simulink library "mssSimulink"  (R2024a)
settings: Solver=ode45  StartTime=0.0  StopTime=10.0  RelTol=1e-3
undefined symbols (not defined in the file): ABC, CN_data, CX_data, CY_data, D, G, Hoerner, K_supply, kt2ms, MA, magnitude, MRB, pathlength, RAO_Amp, RAO_Dir, RAO_Freq, RAO_Phase, RAO_Vel, RAO_yaw_back, RAO_yaw_quant, RAO_yaw_quantization_flag, rho_a, slcm, T_supply, table, vessel, vesselABC
libraries: $bdroot x99, simulink x13
(part 5 of 9)

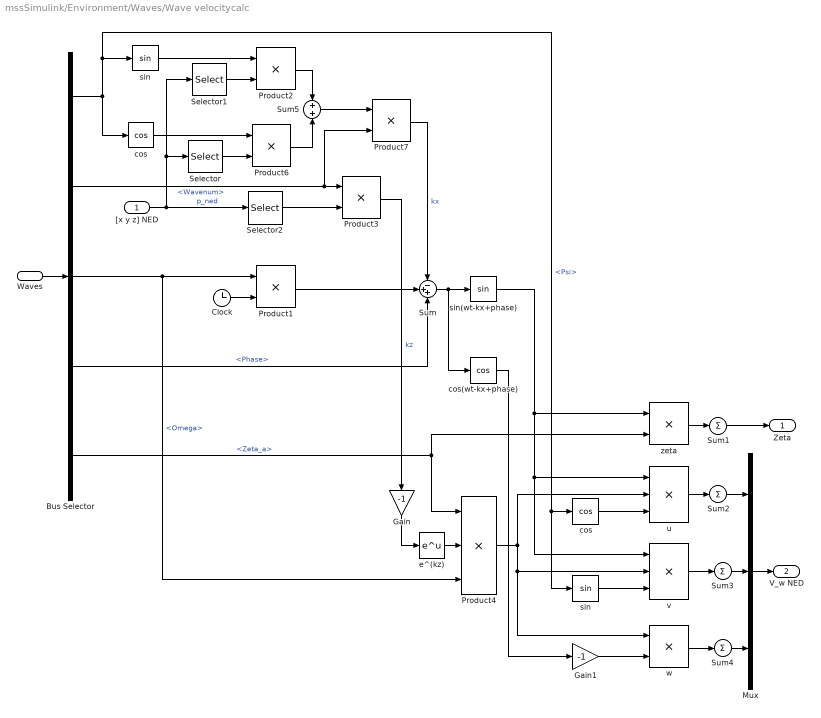
== system mssSimulink/Environment/Waves/Wave velocitycalc ==
  "[x y z] NED" : Inport
  Waves : Inport  Port=2
  Bus Selector : BusSelector  OutputSignals=Psi,Wavenum,Omega,Phase,Zeta_a
  Clock : Clock
  Gain : Gain  Gain=-1  SaturateOnIntegerOverflow=on  OutDataTypeStr=Inherit: Same as input  ParamDataTypeStr=Inherit: Same as input
  Gain1 : Gain  Gain=-1  SaturateOnIntegerOverflow=on  OutDataTypeStr=Inherit: Same as input  ParamDataTypeStr=Inherit: Same as input
  Mux : Mux  Inputs=3
  Product{1..3,6..7} (5 alike) : Product  Inputs=**  SaturateOnIntegerOverflow=on  OutDataTypeStr=Inherit: Same as first input
  Product4 : Product  Inputs=3  SaturateOnIntegerOverflow=on  OutDataTypeStr=Inherit: Same as first input
  Selector : Selector  InputPortWidth=3  IndexOptions=Index vector (dialog)  Indices=1  OutputSizes=1
  Selector1 : Selector  InputPortWidth=3  IndexOptions=Index vector (dialog)  Indices=2  OutputSizes=1
  Selector2 : Selector  InputPortWidth=3  IndexOptions=Index vector (dialog)  Indices=3  OutputSizes=1
  Sum : Sum  Inputs=-++  SaturateOnIntegerOverflow=on
  Sum{1..4} (4 alike) : Sum  Inputs=1  SaturateOnIntegerOverflow=on
  Sum5 : Sum  SaturateOnIntegerOverflow=on
  cos : Trigonometry  Operator=cos
  "cos " : Trigonometry  Operator=cos
  cos(wt-kx+phase) : Trigonometry  Operator=cos
  e^(kz) : Math  SignedPower=on
  sin : Trigonometry
  "sin " : Trigonometry
  sin(wt-kx+phase) : Trigonometry
  u : Product  Inputs=***  SaturateOnIntegerOverflow=on  OutDataTypeStr=Inherit: Same as first input
  v : Product  Inputs=***  SaturateOnIntegerOverflow=on  OutDataTypeStr=Inherit: Same as first input
  w : Product  Inputs=**  SaturateOnIntegerOverflow=on  OutDataTypeStr=Inherit: Same as first input
  zeta : Product  Inputs=**  SaturateOnIntegerOverflow=on  OutDataTypeStr=Inherit: Same as first input
  Zeta : Outport  VectorParamsAs1DForOutWhenUnconnected=off
  V_w NED : Outport  Port=2  VectorParamsAs1DForOutWhenUnconnected=off
  wires:
  Gain1/1 -> w/2
  "cos "/1 -> u/3
  "sin "/1 -> v/3
  Selector2/1 -> Product3/2
  "[x y z] NED"/1 -> Selector/1, Selector1/1, Selector2/1  "p_ned"
  Sum5/1 -> Product7/1
  Product6/1 -> Sum5/2
  Product2/1 -> Sum5/1
  sin/1 -> Product2/1
  Selector1/1 -> Product2/2
  cos/1 -> Product6/1
  Selector/1 -> Product6/2
  Bus Selector/2 -> Product3/1, Product7/2  "<Wavenum>"
  Gain/1 -> e^(kz)/1
  Bus Selector/5 -> Product4/1, zeta/2  "<Zeta_a>"
  Bus Selector/4 -> Sum/3  "<Phase>"
  Bus Selector/3 -> Product4/3, Product1/1  "<Omega>"
  Waves/1 -> Bus Selector/1
  cos(wt-kx+phase)/1 -> Gain1/1
  Product4/1 -> w/1, v/2, u/2
  e^(kz)/1 -> Product4/2
  Product7/1 -> Sum/1  "kx"
  zeta/1 -> Sum1/1
  sin(wt-kx+phase)/1 -> v/1, u/1, zeta/1
  Sum/1 -> cos(wt-kx+phase)/1, sin(wt-kx+phase)/1
  Product1/1 -> Sum/2
  Bus Selector/1 -> sin/1, "cos "/1, "sin "/1, cos/1  "<Psi>"
  Product3/1 -> Gain/1  "kz"
  Sum1/1 -> Zeta/1
  w/1 -> Sum4/1
  u/1 -> Sum2/1
  v/1 -> Sum3/1
  Sum2/1 -> Mux/1
  Sum3/1 -> Mux/2
  Sum4/1 -> Mux/3
  Mux/1 -> V_w NED/1
  Clock/1 -> Product1/2

== system mssSimulink/Environment/Waves/Waves ==
  Bus Creator : BusCreator  Inputs=5
  Omega : Constant  Value=Omega
  Phase : Constant  Value=Phase
  Psi : Constant  Value=Psi
  Wavenum : Constant  Value=Wavenum
  Zeta_a : Constant  Value=Zeta_a
  "wave direction " : Constant  Value=psi_mean
  Waves : Outport  VectorParamsAs1DForOutWhenUnconnected=off
  wave direction : Outport  Port=2  VectorParamsAs1DForOutWhenUnconnected=off
  wires:
  Phase/1 -> Bus Creator/5  "Phase"
  Psi/1 -> Bus Creator/2  "Psi"
  Omega/1 -> Bus Creator/1  "Omega"
  Bus Creator/1 -> Waves/1
  Zeta_a/1 -> Bus Creator/3  "Zeta_a"
  Wavenum/1 -> Bus Creator/4  "Wavenum"
  "wave direction "/1 -> wave direction/1

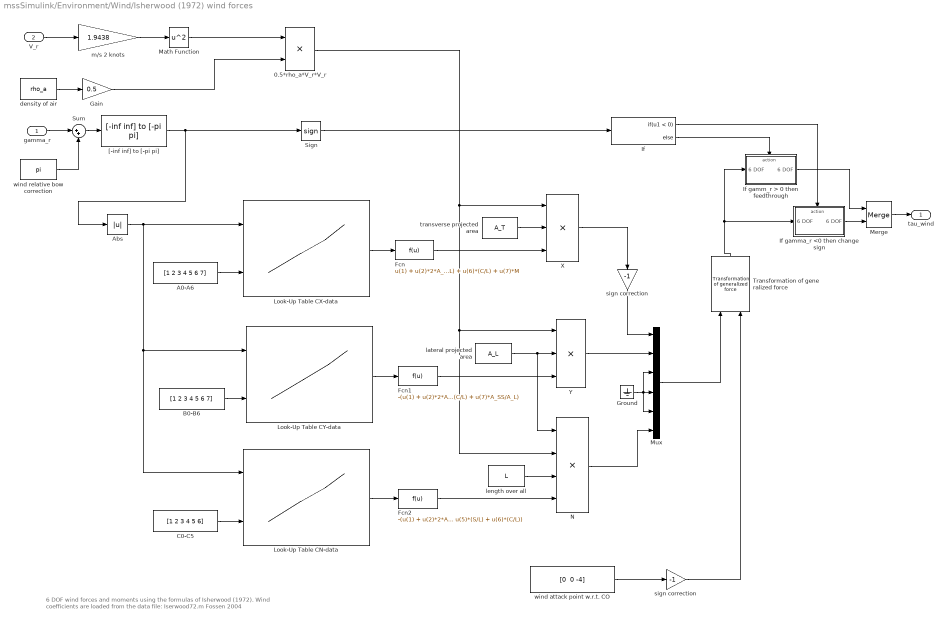
== system mssSimulink/Environment/Wind/Isherwood (1972) wind forces ==
  note: 6 DOF wind forces and moments using the formulas of Isherwood (1972).
      | Wind coefficients are loaded from the data file: Iserwood72.m
      |
      | Fossen 2004
  gamma_r : Inport
  V_r : Inport  Port=2
  0.5*rho_a*V_r*V_r : Product  SaturateOnIntegerOverflow=on  OutDataTypeStr=Inherit: Same as first input
  A0-A6 : Constant  Value=[1 2 3 4 5 6 7]
  Abs : Abs
  B0-B6 : Constant  Value=[1 2 3 4 5 6 7]
  C0-C5 : Constant  Value=[1 2 3 4 5 6]
  Fcn : Fcn  Expr=u(1) + u(2)*2*A_L/L^2 + u(3)*2*A_T/B^2 + u(4)*(L/B) + u(5)*(S/L) + u(6)*(C/L) + u(7)*M
  Fcn1 : Fcn  Expr=-(u(1) + u(2)*2*A_L/L^2 + u(3)*2*A_T/B^2 + u(4)*(L/B) + u(5)*(S/L) + u(6)*(C/L) + u(7)*A_SS/A_L)
  Fcn2 : Fcn  Expr=-(u(1) + u(2)*2*A_L/L^2 + u(3)*2*A_T/B^2 + u(4)*(L/B) + u(5)*(S/L) + u(6)*(C/L))
  Gain : Gain  Gain=0.5  SaturateOnIntegerOverflow=on  OutDataTypeStr=Inherit: Same as input  ParamDataTypeStr=Inherit: Same as input
  Ground : Ground
  If : If  IfExpression=u1 < 0
  If gamm_r > 0 then feedthrough : Subsystem  TreatAsAtomicUnit=on
  If gamma_r <0 then change sign : Subsystem  TreatAsAtomicUnit=on
  Look-Up Table CN-data : Lookup2D  RowIndex=gamma_r_iserwood  ColumnIndex=[1:6]  Table=CN_data  OutDataTypeStr=double  InputSameDT=off
  Look-Up Table CX-data : Lookup2D  RowIndex=gamma_r_iserwood  ColumnIndex=[1:7]  Table=CX_data  OutDataTypeStr=double  InputSameDT=off
  Look-Up Table CY-data : Lookup2D  RowIndex=gamma_r_iserwood  ColumnIndex=[1:7]  Table=CY_data  OutDataTypeStr=double  InputSameDT=off
  Math Function : Math  Operator=square  SignedPower=on
  Merge : Merge
  Mux : Mux  Inputs=6
  N : Product  Inputs=4  SaturateOnIntegerOverflow=on  OutDataTypeStr=Inherit: Same as first input
  Sign : Signum
  Sum : Sum  Inputs=|++  SaturateOnIntegerOverflow=on
  Transformation of gene ralized force : $bdroot/Modelling/Kinematics/Transformation of generalized force
  X : Product  Inputs=3  SaturateOnIntegerOverflow=on  OutDataTypeStr=Inherit: Same as first input
  Y : Product  Inputs=3  SaturateOnIntegerOverflow=on  OutDataTypeStr=Inherit: Same as first input
  "[-inf inf] to [-pi pi]" : $bdroot/Utilities/Math Operations/[-inf inf] to [-pi pi]
  density of air : Constant  Value=rho_a
  lateral projected area : Constant  Value=A_L
  length over all : Constant  Value=L
  m/s 2 knots : Gain  Gain=1.9438  SaturateOnIntegerOverflow=on  OutDataTypeStr=Inherit: Same as input  ParamDataTypeStr=Inherit: Same as input
  sign correction : Gain  Gain=-1  SaturateOnIntegerOverflow=on  OutDataTypeStr=Inherit: Same as input  ParamDataTypeStr=Inherit: Same as input
  "sign correction " : Gain  Gain=-1  SaturateOnIntegerOverflow=on  OutDataTypeStr=Inherit: Same as input  ParamDataTypeStr=Inherit: Same as input
  transverse projected area : Constant  Value=A_T
  wind attack point w.r.t. CO : Constant  Value="[0  0 -4]"
  wind relative bow correction : Constant  Value=pi
  tau_wind : Outport  VectorParamsAs1DForOutWhenUnconnected=off
  wires:
  A0-A6/1 -> Look-Up Table CX-data/2
  Look-Up Table CX-data/1 -> Fcn/1
  B0-B6/1 -> Look-Up Table CY-data/2
  C0-C5/1 -> Look-Up Table CN-data/2
  Look-Up Table CY-data/1 -> Fcn1/1
  Look-Up Table CN-data/1 -> Fcn2/1
  gamma_r/1 -> Sum/1
  Fcn/1 -> X/3
  Fcn1/1 -> Y/3
  Fcn2/1 -> N/4
  density of air/1 -> Gain/1
  V_r/1 -> m/s 2 knots/1
  Math Function/1 -> 0.5*rho_a*V_r*V_r/1
  Gain/1 -> 0.5*rho_a*V_r*V_r/2
  0.5*rho_a*V_r*V_r/1 -> X/1, Y/1, N/2
  transverse projected area/1 -> X/2
  X/1 -> sign correction/1
  lateral projected area/1 -> Y/2, N/1
  Y/1 -> Mux/2
  N/1 -> Mux/6
  length over all/1 -> N/3
  m/s 2 knots/1 -> Math Function/1
  Abs/1 -> Look-Up Table CX-data/1, Look-Up Table CY-data/1, Look-Up Table CN-data/1
  Transformation of gene ralized force/1 -> If gamma_r <0 then change sign/1(6 DOF), If gamm_r > 0 then feedthrough/1(6 DOF)
  If/2 -> If gamm_r > 0 then feedthrough/Action
  If/1 -> If gamma_r <0 then change sign/Action
  If gamma_r <0 then change sign/1("6 DOF  ") -> Merge/2
  If gamm_r > 0 then feedthrough/1("6 DOF  ") -> Merge/1
  Sign/1 -> If/1
  wind attack point w.r.t. CO/1 -> "sign correction "/1
  "sign correction "/1 -> Transformation of gene ralized force/2
  Merge/1 -> tau_wind/1
  Mux/1 -> Transformation of gene ralized force/1
  Ground/1 -> Mux/3, Mux/4, Mux/5
  wind relative bow correction/1 -> Sum/2
  Sum/1 -> "[-inf inf] to [-pi pi]"/1
  "[-inf inf] to [-pi pi]"/1 -> Abs/1, Sign/1
  sign correction/1 -> Mux/1

== system mssSimulink/Environment/Wind/Relative wind speed and angle of attack ==
  note: v
  beta_Vw : Inport
  V_w : Inport  Port=2
  psi : Inport  Port=3
  u : Inport  Port=4
  v : Inport  Port=5
  Magnitude Squared : Math  Operator=magnitude^2
  Magnitude Squared1 : Math  Operator=magnitude^2
  Product : Product
  Product1 : Product
  Sqrt : Sqrt
  Sum : Sum  Inputs=|+-
  Sum1 : Sum  Inputs=|-+
  Sum2 : Sum  Inputs=|-+
  Sum3 : Sum  Inputs=|++
  Trigonometric Function : Trigonometry
  Trigonometric Function1 : Trigonometry  Operator=cos
  Trigonometric Function2 : Trigonometry  Operator=atan2
  gamma_r : Outport
  V_r : Outport  Port=2
  wires:
  V_w/1 -> Product1/1, Product/1
  beta_Vw/1 -> Sum/1
  psi/1 -> Sum/2
  Sum/1 -> Trigonometric Function/1, Trigonometric Function1/1
  Trigonometric Function1/1 -> Product/2
  Trigonometric Function/1 -> Product1/2
  Product/1 -> Sum2/1  "u_w"
  Product1/1 -> Sum1/1  "v_w"
  v/1 -> Sum1/2
  Sum1/1 -> Trigonometric Function2/1, Magnitude Squared1/1  "v_r"
  u/1 -> Sum2/2  "u"
  Sum2/1 -> Trigonometric Function2/2, Magnitude Squared/1
  Magnitude Squared/1 -> Sum3/1
  Magnitude Squared1/1 -> Sum3/2
  Sum3/1 -> Sqrt/1
  Sqrt/1 -> V_r/1
  Trigonometric Function2/1 -> gamma_r/1

== system mssSimulink/Environment/Wind/Wind ==
  Gust : Constant  Value=Par_Wind_gust
  Mean angle : Constant  Value=Par_Wind_angle
  Mean velocity : Constant  Value=Par_Wind_V
  Slowly-varying wind : Subsystem  mask(Slowly-varying wind){Par_Wind_sample_time=Par_Wind_sample_time, Par_Wind_speed_T=Par_Wind_speed_T, Par_Wind_angle_T=Par_Wind_angle_T, Par_Wind_speed_noise_pow=Par_Wind_speed_noise_pow, Par_Wind_angle_noise_pow=Par_Wind_angle_noise_pow, Par_Wind_speed_rand_max=Par_Wind_speed_rand_max, Par_Wind_angle_rand_max=Par_Wind_angle_rand_max, Par_Wind_speed_seed=Par_Wind_speed_seed, Par_Wind_angle_seed=Par_Wind_angle_seed}
      mask prompts: Par_Wind_sample_time "Wind sample time [s]"; Par_Wind_speed_T "Wind speed time constant [s]"; Par_Wind_angle_T "Wind angle time constant [s]"; Par_Wind_speed_noise_pow "Wind speed noise power"; Par_Wind_angle_noise_pow "Wind angle noise power"; Par_Wind_speed_rand_max "Wind speed saturation [m/s] (max random variation about mean)"; Par_Wind_angle_rand_max "Wind angle saturation [rad] (max random variation about mean)"; Par_Wind_speed_seed "Wind speed random seed"; Par_Wind_angle_seed "Wind angle random seed"
      mask help:
      | Generate slowly varying wind speed and direction based on random processes.
      |
      | stochastic = 0  gives constant mean wind speed and direction
      | stochastic = 1  gives stochastic mean wind speed and direction
      mask Help:
      | Generate slowly varying wind speed and direction based on random processes.<br>
      | <br>
      | stochastic = 0 gives constant mean wind direction and speed,<br>
      | stochastic = 1 gives stochastic mean wind direction and speed<br>
      | <br>
      | <p>The randomness of the mean speed and angle can be limited by two saturation
      | parameters, which define the maximum random deviation from the mean value.<br>
  Slowlyvar : Constant  Value=Par_Wind_slowlyvar
  Sum : Sum  Inputs=++|  SaturateOnIntegerOverflow=on
  Sum1 : Sum  Inputs=+++  SaturateOnIntegerOverflow=on
  Wind gust : Subsystem  mask(Wind gust){Par_Wind_spectrum_type=Par_Wind_spectrum_type, Par_Wind_phase_seed=Par_Wind_phase_seed, Par_Wind_kappa_H=Par_Wind_kappa_H, Par_Wind_L=Par_Wind_L, Par_Wind_z=Par_Wind_z, Par_Wind_minfreq=Par_Wind_minfreq, Par_Wind_maxfreq=Par_Wind_maxfreq, Par_Wind_nfreq=Par_Wind_nfreq}
      mask prompts: Par_Wind_spectrum_type "Spectrum type"; Par_Wind_phase_seed "Wind gust phase seed"; Par_Wind_kappa_H "Sea surface drag coefficient for Harris wind spectrum (0.0026)"; Par_Wind_L "Scaling length for Harris wind spectrum (1800)"; Par_Wind_z "Height over water surface, for NORSOK spectrum"; Par_Wind_minfreq "Minimum frequency in gust [Hz] (1E-4)"; Par_Wind_maxfreq "Maximum frequency in gust [Hz] (0.1)"; Par_Wind_nfreq "Number of frequency components"
      mask help:
      | Calculate the wind gust according to one of two gust spectra:
      |
      | 1) Harris (based on measurements over land)
      | 2) NORSOK (based on measurements from the North Sea)
      |
      | The gust from the Harris spectrum is not influenced by the heigth over the sea surface, whereas the gust from the NORSOK spectrum is.
  angle : Outport  VectorParamsAs1DForOutWhenUnconnected=off
  speed : Outport  Port=2  VectorParamsAs1DForOutWhenUnconnected=off
  wires:
  Gust/1 -> Wind gust/Enable
  Slowlyvar/1 -> Slowly-varying wind/Enable
  Slowly-varying wind/1(angle) -> Sum/2
  Mean velocity/1 -> Wind gust/1(u10), Sum1/3
  Mean angle/1 -> Sum/1
  Sum/1 -> angle/1
  Wind gust/1(Gust) -> Sum1/2
  Slowly-varying wind/2(speed) -> Sum1/1
  Sum1/1 -> speed/1

== system mssSimulink/Guidance/Waypoint guidance block/Stop vessel ==
  theta : Inport
  If endpoint1 : If  IfExpression=u1 > size(table,2)
  Merge : Merge
  Model Info : simulink/Model-Wide Utilities/Model Info  Frame=on  DisplayStringWithTags=|  HorizontalTextAlignment=Center  LeftAlignmentValue=0.5
      | Stop vessel
      | This subsystem performs an action when
      | the vessel reaches the last waypoint. The 
      | simultation is either stopped, or the desired 
      | speed is set to zero.
      | Author: Jorgen Corneliussen
      | Modified: %<ModifiedDate>
      | Version: %<ModelVersion>
  Reached endpoint : Subsystem  TreatAsAtomicUnit=on
  Still travelling : Subsystem  TreatAsAtomicUnit=on
  stopsignal : Outport  VectorParamsAs1DForOutWhenUnconnected=off
  wires:
  Still travelling/1(one) -> Merge/2
  theta/1 -> If endpoint1/1
  If endpoint1/1 -> Reached endpoint/Action
  Reached endpoint/1(zero) -> Merge/1
  Merge/1 -> stopsignal/1
  If endpoint1/2 -> Still travelling/Action

== system mssSimulink/Guidance/Waypoint guidance block/Thetacomputation ==
  theta : Inport
  5th order algorithm : Subsystem  TreatAsAtomicUnit=on
  Constant1 : Constant  Value=method
  Cubic splines : Subsystem  TreatAsAtomicUnit=on
  If endpoint1 : If  IfExpression=u1 == 1
  Model Info : simulink/Model-Wide Utilities/Model Info  Frame=on  DisplayStringWithTags=|  HorizontalTextAlignment=Center  LeftAlignmentValue=0.5
      | Thetacomputation
      | This subsystem returns a vector containing 
      | different orders of theta.
      | If cubic splines is used, the system returns:
      | [th^3 th^2 th 1]
      | If the 5th order polynomial is used, it returns:
      | [th^5 th^4 th^3 th^2 th 1]
      | Author: Jorgen Corneliussen
      | Modified: %<ModifiedDate>
      | Version: %<ModelVersion>
  Multiport Switch : MultiPortSwitch  Inputs=2  InputSameDT=off
  Selector : Selector  InputPortWidth=6  IndexOptions=Index vector (dialog)  Indices=[1:size(table,1)/8]  OutputSizes=1
  thetavector : Outport  VectorParamsAs1DForOutWhenUnconnected=off
  wires:
  If endpoint1/1 -> Cubic splines/Action  "cubic"
  If endpoint1/2 -> 5th order algorithm/Action
  Constant1/1 -> If endpoint1/1, Multiport Switch/1
  theta/1 -> 5th order algorithm/1(theta), Cubic splines/1(theta)
  5th order algorithm/1(theta_vector) -> Multiport Switch/3
  Selector/1 -> thetavector/1
  Cubic splines/1(theta_vector) -> Multiport Switch/2
  Multiport Switch/1 -> Selector/1

== system mssSimulink/Guidance/Waypoint guidance block/vs_calculations ==
  ud : Inport
  ud_dot : Inport  Port=2
  xd_theta : Inport  Port=3
  yd_theta : Inport  Port=4
  xd_theta_2 : Inport  Port=5
  yd_theta_2 : Inport  Port=6
  Model Info : simulink/Model-Wide Utilities/Model Info  Frame=on  DisplayStringWithTags=|  HorizontalTextAlignment=Center  LeftAlignmentValue=0.5
      | vs_calculations
      | This subsystem returns a vector containing 
      | the  speed assignment along the path.
      | The vector contains the desired speed, and 
      | the derivative of the desired speed with regards
      |  to theta and with regards to time.
      | Author: Jorgen Corneliussen
      | Modified: %<ModifiedDate>
      | Version: %<ModelVersion>
  vs_calc : Subsystem
  vs_t_calc : Subsystem
  vs_theta_calc : Subsystem
  vs : Outport  VectorParamsAs1DForOutWhenUnconnected=off
  vs_theta : Outport  Port=2  VectorParamsAs1DForOutWhenUnconnected=off
  vs_t : Outport  Port=3  VectorParamsAs1DForOutWhenUnconnected=off
  wires:
  vs_calc/1(vs) -> vs/1  "vs"
  vs_theta_calc/1(vs_theta) -> vs_theta/1  "vs_theta"
  vs_t_calc/1(vs_t) -> vs_t/1  "vs_t"
  ud/1 -> vs_calc/1(ud), vs_theta_calc/5(ud)
  ud_dot/1 -> vs_t_calc/3(ud_dot)
  xd_theta/1 -> vs_calc/2(xd_theta), vs_theta_calc/1(xd_theta), vs_t_calc/1(xd_theta)
  yd_theta/1 -> vs_calc/3(yd_theta), vs_theta_calc/3(yd_theta), vs_t_calc/2(yd_theta)
  xd_theta_2/1 -> vs_theta_calc/2(xd_theta_2)
  yd_theta_2/1 -> vs_theta_calc/4(yd_theta_2)

== system mssSimulink/Hydrodynamics/6-DOF maneuvering model (unified model with fluid memory)/Model Info1 ==
  EmptySubsystem : Subsystem

== system mssSimulink/Hydrodynamics/Cross-flow drag and surge resistance/Cross-flow drag trapezoidal integration ==
  N : Inport
  dx : Inport  Port=2
  v_r : Inport  Port=3
  r : Inport  Port=4
  Abs : Abs
  For Iterator : ForIterator  ResetStates=reset  IterationSource=external  IterationVariableDataType=double
  If i=1 or i=N : If  NumInputs=2  IfExpression=u1 == 1 | u1 == u2
  Lpp/2 : Constant  Value=Lpp/2
  Merge : Merge
  Product : Product  Inputs=**  SaturateOnIntegerOverflow=on  OutDataTypeStr=Inherit: Same as first input
  Product1 : Product  Inputs=**  SaturateOnIntegerOverflow=on  OutDataTypeStr=Inherit: Same as first input
  Product3 : Product  SaturateOnIntegerOverflow=on  OutDataTypeStr=Inherit: Same as first input
  Product4 : Product  SaturateOnIntegerOverflow=on  OutDataTypeStr=Inherit: Same as first input
  Sum : Sum  Inputs=|++  InputSameDT=on  SaturateOnIntegerOverflow=on  OutDataTypeStr=Inherit: Same as first input
  Sum1 : Sum  Inputs=++|  SaturateOnIntegerOverflow=on
  Sum2 : Sum  Inputs=|++  InputSameDT=on  SaturateOnIntegerOverflow=on  OutDataTypeStr=Inherit: Same as first input
  Sum3 : Sum  Inputs=+-|  InputSameDT=on  SaturateOnIntegerOverflow=on  OutDataTypeStr=Inherit: Same as first input
  Sum4 : Sum  Inputs=+-|  InputSameDT=on  SaturateOnIntegerOverflow=on  OutDataTypeStr=Inherit: Same as first input
  constant : Constant
  memory1 : Memory  InheritSampleTime=on
  memory2 : Memory  InheritSampleTime=on
  multiply with 0.5 : Subsystem  TreatAsAtomicUnit=on
  multiply with 1 : Subsystem  TreatAsAtomicUnit=on
  x * r : Product  SaturateOnIntegerOverflow=on  OutDataTypeStr=Inherit: Same as first input
  sum1 : Outport
  sum2 : Outport  Port=2
  wires:
  For Iterator/1 -> If i=1 or i=N/1, Sum4/1  "i"
  N/1 -> For Iterator/1, If i=1 or i=N/2
  Sum1/1 -> Product3/2, Abs/1
  x * r/1 -> Sum1/2
  Abs/1 -> Product3/1
  v_r/1 -> Sum1/1
  Sum/1 -> sum1/1, memory1/1
  memory1/1 -> Sum/1
  Sum2/1 -> sum2/1, memory2/1
  memory2/1 -> Sum2/1
  dx/1 -> Product1/1, Product/1  "dx"
  Lpp/2/1 -> Sum3/2
  Product1/1 -> Sum3/1
  Sum4/1 -> Product1/2  "i-1"
  constant/1 -> Sum4/2
  Sum3/1 -> x * r/2, Product4/2  "x"
  r/1 -> x * r/1
  Product4/1 -> Sum2/2
  Product3/1 -> Product/2
  Product/1 -> multiply with 1/1(In1), multiply with 0.5/1(In1)
  If i=1 or i=N/1 -> multiply with 0.5/Action
  If i=1 or i=N/2 -> multiply with 1/Action
  multiply with 0.5/1(Out1) -> Merge/1
  multiply with 1/1(Out1) -> Merge/2
  Merge/1 -> Sum/2, Product4/1

== system mssSimulink/Hydrodynamics/Fluid memory effetcs/heave ==
  nu : Inport
  Selector : Selector  InputPortWidth=6  IndexOptions=Index vector (dialog)  Indices=[1]  OutputSizes=1
  Selector1 : Selector  InputPortWidth=6  IndexOptions=Index vector (dialog)  Indices=[3]  OutputSizes=1
  Selector2 : Selector  InputPortWidth=6  IndexOptions=Index vector (dialog)  Indices=[5]  OutputSizes=1
  u : Outport
  w : Outport  Port=2
  q : Outport  Port=3
  wires:
  nu/1 -> Selector/1, Selector1/1, Selector2/1
  Selector/1 -> u/1
  Selector1/1 -> w/1
  Selector2/1 -> q/1

== system mssSimulink/Hydrodynamics/Fluid memory effetcs/pitch ==
  nu : Inport
  Selector : Selector  InputPortWidth=6  IndexOptions=Index vector (dialog)  Indices=[1]  OutputSizes=1
  Selector1 : Selector  InputPortWidth=6  IndexOptions=Index vector (dialog)  Indices=[3]  OutputSizes=1
  Selector2 : Selector  InputPortWidth=6  IndexOptions=Index vector (dialog)  Indices=[5]  OutputSizes=1
  u : Outport
  w : Outport  Port=2
  q : Outport  Port=3
  wires:
  nu/1 -> Selector/1, Selector1/1, Selector2/1
  Selector/1 -> u/1
  Selector1/1 -> w/1
  Selector2/1 -> q/1

== system mssSimulink/Hydrodynamics/Fluid memory effetcs/roll ==
  nu : Inport
  Selector : Selector  InputPortWidth=6  IndexOptions=Index vector (dialog)  Indices=[2]  OutputSizes=1
  Selector1 : Selector  InputPortWidth=6  IndexOptions=Index vector (dialog)  Indices=[4]  OutputSizes=1
  Selector2 : Selector  InputPortWidth=6  IndexOptions=Index vector (dialog)  Indices=[6]  OutputSizes=1
  v : Outport
  p : Outport  Port=2
  r : Outport  Port=3
  wires:
  nu/1 -> Selector/1, Selector1/1, Selector2/1
  Selector/1 -> v/1
  Selector1/1 -> p/1
  Selector2/1 -> r/1

== system mssSimulink/Hydrodynamics/Fluid memory effetcs/surge ==
  nu : Inport
  Selector : Selector  InputPortWidth=6  IndexOptions=Index vector (dialog)  Indices=[1]  OutputSizes=1
  Selector1 : Selector  InputPortWidth=6  IndexOptions=Index vector (dialog)  Indices=[3]  OutputSizes=1
  Selector2 : Selector  InputPortWidth=6  IndexOptions=Index vector (dialog)  Indices=[5]  OutputSizes=1
  u : Outport
  w : Outport  Port=2
  q : Outport  Port=3
  wires:
  nu/1 -> Selector/1, Selector1/1, Selector2/1
  Selector/1 -> u/1
  Selector1/1 -> w/1
  Selector2/1 -> q/1

== system mssSimulink/Hydrodynamics/Fluid memory effetcs/sway ==
  nu : Inport
  Selector : Selector  InputPortWidth=6  IndexOptions=Index vector (dialog)  Indices=[2]  OutputSizes=1
  Selector1 : Selector  InputPortWidth=6  IndexOptions=Index vector (dialog)  Indices=[4]  OutputSizes=1
  Selector2 : Selector  InputPortWidth=6  IndexOptions=Index vector (dialog)  Indices=[6]  OutputSizes=1
  v : Outport
  p : Outport  Port=2
  r : Outport  Port=3
  wires:
  nu/1 -> Selector/1, Selector1/1, Selector2/1
  Selector/1 -> v/1
  Selector1/1 -> p/1
  Selector2/1 -> r/1

== system mssSimulink/Hydrodynamics/Fluid memory effetcs/yaw ==
  nu : Inport
  Selector : Selector  InputPortWidth=6  IndexOptions=Index vector (dialog)  Indices=[2]  OutputSizes=1
  Selector1 : Selector  InputPortWidth=6  IndexOptions=Index vector (dialog)  Indices=[4]  OutputSizes=1
  Selector2 : Selector  InputPortWidth=6  IndexOptions=Index vector (dialog)  Indices=[6]  OutputSizes=1
  v : Outport
  p : Outport  Port=2
  r : Outport  Port=3
  wires:
  nu/1 -> Selector/1, Selector1/1, Selector2/1
  Selector/1 -> v/1
  Selector1/1 -> p/1
  Selector2/1 -> r/1

== system mssSimulink/Hydrodynamics/Motion RAO (U=0)/6DOF rotation matrix in yaw ==
  psi : Inport
  V : Inport  Port=2
  Mux1 : Mux  Inputs=2
  Rotation matrix in yaw : $bdroot/Modelling/Kinematics/Rotation matrix in yaw 
  Selector : Selector  InputPortWidth=6  IndexOptions=Index vector (dialog)  Indices=[4 5 6]  OutputSizes=1
  Selector2 : Selector  InputPortWidth=6  IndexOptions=Index vector (dialog)  Indices=[1 2 3]  OutputSizes=1
  R(psi)*V : Outport
  wires:
  Rotation matrix in yaw/1 -> Mux1/1
  V/1 -> Selector/1, Selector2/1
  psi/1 -> Rotation matrix in yaw/1
  Selector2/1 -> Rotation matrix in yaw/2
  Mux1/1 -> R(psi)*V/1
  Selector/1 -> Mux1/2

== system mssSimulink/Hydrodynamics/Motion RAO (U=0)/Output smoothing ==
  eta_h WF : Inport
  "nu WF " : Inport  Port=2
  "nu_dot WF " : Inport  Port=3
  nu_dot rate : Inport  Port=4
  Output smoothing flag : Constant  Value=RAO_smoothing_flag
  Signal smoothing 1 : $bdroot/Modelling/Environmental Loads/Utilities/Signal smoothing
  Signal smoothing 2 : $bdroot/Modelling/Environmental Loads/Utilities/Signal smoothing
  Signal smoothing 3 : $bdroot/Modelling/Environmental Loads/Utilities/Signal smoothing
  Switch1 : Switch  Threshold=0.5  SaturateOnIntegerOverflow=off  InputSameDT=off
  Switch2 : Switch  Threshold=0.5  SaturateOnIntegerOverflow=off  InputSameDT=off
  Switch3 : Switch  Threshold=0.5  SaturateOnIntegerOverflow=off  InputSameDT=off
  "eta_h WF " : Outport
  nu WF : Outport  Port=2
  nu_dot WF : Outport  Port=3
  wires:
  Switch1/1 -> nu WF/1
  Switch3/1 -> nu_dot WF/1
  nu_dot rate/1 -> Signal smoothing 3/2
  Signal smoothing 3/1 -> Switch3/1
  "nu_dot WF "/1 -> Switch3/3, Signal smoothing 2/2, Signal smoothing 3/1
  Switch2/1 -> "eta_h WF "/1
  Signal smoothing 2/1 -> Switch1/1
  "nu WF "/1 -> Switch1/3, Signal smoothing 1/2, Signal smoothing 2/1
  eta_h WF/1 -> Switch2/3, Signal smoothing 1/1
  Signal smoothing 1/1 -> Switch2/1
  Output smoothing flag/1 -> Switch3/2, Switch1/2, Switch2/2

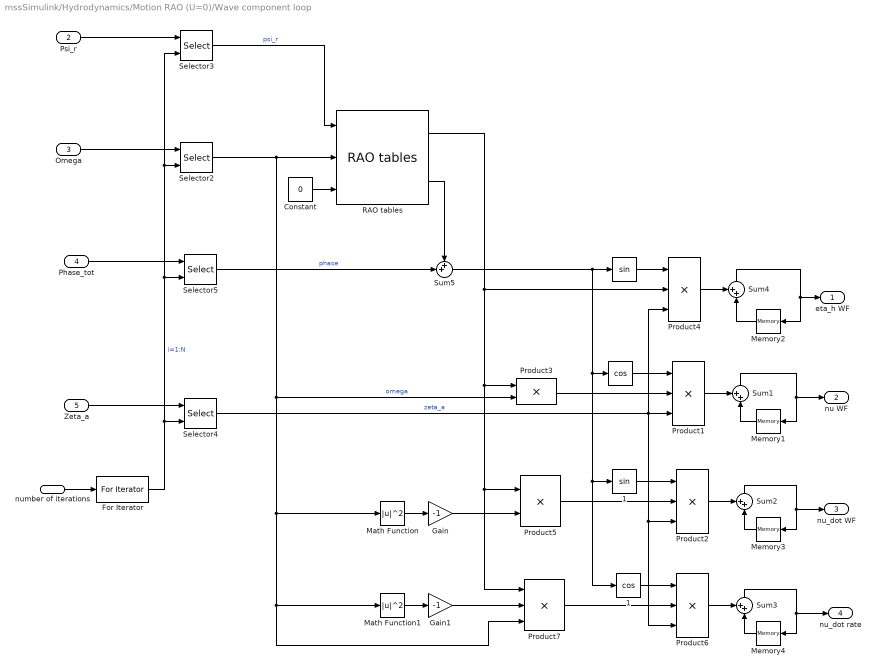
== system mssSimulink/Hydrodynamics/Motion RAO (U=0)/Wave component loop ==
  number of iterations : Inport
  Psi_r : Inport  Port=2
  Omega : Inport  Port=3
  Phase_tot : Inport  Port=4
  Zeta_a : Inport  Port=5
  "              " : Trigonometry  Operator=cos
  "                " : Trigonometry
  "                1" : Trigonometry
  "              1" : Trigonometry  Operator=cos
  Constant : Constant  Value=0
  For Iterator : ForIterator  ResetStates=reset  IterationSource=external  IterationVariableDataType=double
  Gain : Gain  Gain=-1  SaturateOnIntegerOverflow=on  OutDataTypeStr=Inherit: Same as input  ParamDataTypeStr=Inherit: Same as input
  Gain1 : Gain  Gain=-1  SaturateOnIntegerOverflow=on  OutDataTypeStr=Inherit: Same as input  ParamDataTypeStr=Inherit: Same as input
  Math Function : Math  Operator=magnitude^2  SignedPower=on
  Math Function1 : Math  Operator=magnitude^2  SignedPower=on
  Memory{1..4} (4 alike) : Memory  InitialCondition=[0 0 0 0 0 0]'  InheritSampleTime=on
  Product{1..2,4,6} (4 alike) : Product  Inputs=3  SaturateOnIntegerOverflow=on  OutDataTypeStr=Inherit: Same as first input
  Product3 : Product  Inputs=**  SaturateOnIntegerOverflow=on  OutDataTypeStr=Inherit: Same as first input
  Product5 : Product  Inputs=**  SaturateOnIntegerOverflow=on  OutDataTypeStr=Inherit: Same as first input
  Product7 : Product  Inputs=***  SaturateOnIntegerOverflow=on  OutDataTypeStr=Inherit: Same as first input
  "RAO tables " : $bdroot/Modelling/Environmental Loads/Utilities/RAO tables  RAO_Freq=RAO_Freq  RAO_Dir=RAO_Dir  RAO_Vel=RAO_Vel  RAO_Amp=RAO_Amp  RAO_Phase=RAO_Phase
  Selector{2..5} (4 alike) : Selector  IndexOptions=Index vector (port)  Indices=[1 3]  OutputSizes=1
  Sum{1..5} (5 alike) : Sum  Inputs=++|  SaturateOnIntegerOverflow=on
  eta_h WF : Outport
  nu WF : Outport  Port=2
  nu_dot WF : Outport  Port=3
  nu_dot rate : Outport  Port=4
  wires:
  Product7/1 -> Product6/2
  "              1"/1 -> Product6/1
  Math Function1/1 -> Gain1/1
  Gain1/1 -> Product7/2
  Memory4/1 -> Sum3/2
  Product6/1 -> Sum3/1
  Sum3/1 -> Memory4/1, nu_dot rate/1
  Selector3/1 -> "RAO tables "/1  "psi_r"
  Selector2/1 -> Product7/3, Math Function1/1, Math Function/1, Product3/2, "RAO tables "/2  "omega"
  Selector5/1 -> Sum5/2  "phase"
  Product4/1 -> Sum4/1
  Memory2/1 -> Sum4/2
  Sum4/1 -> eta_h WF/1, Memory2/1
  number of iterations/1 -> For Iterator/1
  Omega/1 -> Selector2/1
  For Iterator/1 -> Selector3/2, Selector2/2, Selector5/2, Selector4/2  "i=1:N"
  Psi_r/1 -> Selector3/1
  Constant/1 -> "RAO tables "/3
  "RAO tables "/1 -> Product4/2, Product7/1, Product5/1, Product3/1
  "RAO tables "/2 -> Sum5/1
  Phase_tot/1 -> Selector5/1
  Zeta_a/1 -> Selector4/1
  Sum5/1 -> "                "/1, "              1"/1, "                1"/1, "              "/1
  "                "/1 -> Product4/1
  Selector4/1 -> Product6/3, Product2/3, Product1/3, Product4/3  "zeta_a"
  "              "/1 -> Product1/1
  Memory1/1 -> Sum1/2
  Sum1/1 -> nu WF/1, Memory1/1
  Product1/1 -> Sum1/1
  Memory3/1 -> Sum2/2
  Product2/1 -> Sum2/1
  Sum2/1 -> nu_dot WF/1, Memory3/1
  "                1"/1 -> Product2/1
  Math Function/1 -> Gain/1
  Gain/1 -> Product5/2
  Product5/1 -> Product2/2
  Product3/1 -> Product1/2

== system mssSimulink/Hydrodynamics/WD for heading1/Wave component loop ==
  number of iterations : Inport
  Psi_r : Inport  Port=2
  Omega : Inport  Port=3
  Zeta_a : Inport  Port=4
  U : Inport  Port=5
  Direct Lookup Table (n-D) Beta : LookupNDDirect  NumberOfTableDimensions=1  Table=vessel.headings
  Direct Lookup Table (n-D) Velocity : LookupNDDirect  NumberOfTableDimensions=1  Table=RAO_Vel
  For Iterator : ForIterator  ResetStates=reset  IterationSource=external  IterationVariableDataType=double
  Memory1 : Memory  InitialCondition=[0 0 0 0 0 0]'  InheritSampleTime=on
  Prelookup1 : PreLookup  BreakpointsData=vessel.headings  OutputSelection=Index only  IndexSearchMethod=Evenly spaced points  BeginIndexSearchUsingPreviousIndexResult=on
  Prelookup2 : PreLookup  BreakpointsData=RAO_Vel  OutputSelection=Index only  IndexSearchMethod=Linear search  BeginIndexSearchUsingPreviousIndexResult=on
  Product3 : Product  Inputs=3  SaturateOnIntegerOverflow=on  OutDataTypeStr=Inherit: Same as first input
  Selector2 : Selector  IndexOptions=Index vector (port)  Indices=[1 3]  OutputSizes=1
  Selector3 : Selector  IndexOptions=Index vector (port)  Indices=[1 3]  OutputSizes=1
  Selector4 : Selector  IndexOptions=Index vector (port)  Indices=[1 3]  OutputSizes=1
  Sum1 : Sum  Inputs=++|  SaturateOnIntegerOverflow=on
  WD RAO tables : Subsystem  mask(RAO table lookup){}
      mask help:
      | Perform 3D table lookup in 6DOF RAO amplitudes and phases, using the relative wave heading psi_r, wave frequency omega and vessel velocity vel as inputs. See documentation of the Motion RAO block or Force RAO block for details. A warning is issued if the input is outside the range spanned by the RAOs.
      |
      | Author: Oyvind N. Smogeli and Thor I. Fossen, 2005-05-03
  "[-inf inf] to [-pi pi] " : $bdroot/Utilities/Math Operations/[-inf inf] to [-pi pi]
  "[-pi pi] to [0 2pi]" : Subsystem  mask([-inf inf] to [-pi pi]){}
      mask help: Converts an angle in rad to (-pi pi)
  tau_WD : Outport
  wires:
  Selector4/1 -> Product3/2, Product3/3  "zeta_a"
  Zeta_a/1 -> Selector4/1
  U/1 -> Prelookup2/1
  Psi_r/1 -> Selector3/1
  Omega/1 -> Selector2/1
  number of iterations/1 -> For Iterator/1
  Selector3/1 -> "[-inf inf] to [-pi pi] "/1  "psi_r"
  Sum1/1 -> Memory1/1, tau_WD/1
  Memory1/1 -> Sum1/2
  Product3/1 -> Sum1/1
  "[-pi pi] to [0 2pi]"/1(0<y<2pi) -> Prelookup1/1
  Selector2/1 -> WD RAO tables/2(w)  "omega"
  For Iterator/1 -> Selector3/2, Selector4/2, Selector2/2  "i=1:N"
  "[-inf inf] to [-pi pi] "/1 -> "[-pi pi] to [0 2pi]"/1(x [-pi pi])
  Prelookup1/1 -> Direct Lookup Table (n-D) Beta/1
  Direct Lookup Table (n-D) Beta/1 -> WD RAO tables/1(beta)
  Prelookup2/1 -> Direct Lookup Table (n-D) Velocity/1
  Direct Lookup Table (n-D) Velocity/1 -> WD RAO tables/3(U)
  WD RAO tables/1(amp) -> Product3/1

== system mssSimulink/Hydrodynamics/Wave drift (U=0)/psi1 ==
  k : Inport
  0 or 1 : Inport  Port=2
  Gain1 : Gain  Gain=20
  Gain2 : Gain  Gain=10
  Product : Product  RndMeth=Zero
  Sum7 : Sum  Inputs=-+|
  Sum8 : Sum  Inputs=++|
  const : Constant  Value=18
  psi : Outport
  wires:
  const/1 -> Sum7/2
  Sum7/1 -> Gain1/1
  Gain1/1 -> Product/1
  Product/1 -> Sum8/2
  Gain2/1 -> Sum8/1
  k/1 -> Sum7/1, Gain2/1
  Sum8/1 -> psi/1
  0 or 1/1 -> Product/2

== system mssSimulink/Hydrodynamics/Wave drift (U=0)/psi2 ==
  k : Inport
  0 or 1 : Inport  Port=2
  Gain1 : Gain  Gain=20
  Gain2 : Gain  Gain=10
  Product : Product  RndMeth=Zero
  Sum7 : Sum  Inputs=-+|
  Sum8 : Sum  Inputs=++|
  const : Constant  Value=18
  psi : Outport
  wires:
  const/1 -> Sum7/2
  Sum7/1 -> Gain1/1
  Gain1/1 -> Product/1
  Product/1 -> Sum8/2
  Gain2/1 -> Sum8/1
  k/1 -> Sum7/1, Gain2/1
  Sum8/1 -> psi/1
  0 or 1/1 -> Product/2

== system mssSimulink/Hydrodynamics/Wave loads (U=0)/psi1 ==
  k : Inport
  0 or 1 : Inport  Port=2
  Gain1 : Gain  Gain=20
  Gain2 : Gain  Gain=10
  Product : Product  RndMeth=Zero
  Sum7 : Sum  Inputs=-+|
  Sum8 : Sum  Inputs=++|
  const : Constant  Value=18
  psi : Outport
  wires:
  0 or 1/1 -> Product/2
  Sum8/1 -> psi/1
  k/1 -> Gain2/1, Sum7/1
  Gain2/1 -> Sum8/1
  Product/1 -> Sum8/2
  Gain1/1 -> Product/1
  Sum7/1 -> Gain1/1
  const/1 -> Sum7/2

== system mssSimulink/Hydrodynamics/Wave loads (U=0)/psi2 ==
  k : Inport
  0 or 1 : Inport  Port=2
  Gain1 : Gain  Gain=20
  Gain2 : Gain  Gain=10
  Product : Product  RndMeth=Zero
  Sum7 : Sum  Inputs=-+|
  Sum8 : Sum  Inputs=++|
  const : Constant  Value=18
  psi : Outport
  wires:
  0 or 1/1 -> Product/2
  Sum8/1 -> psi/1
  k/1 -> Gain2/1, Sum7/1
  Gain2/1 -> Sum8/1
  Product/1 -> Sum8/2
  Gain1/1 -> Product/1
  Sum7/1 -> Gain1/1
  const/1 -> Sum7/2

== system mssSimulink/Hydrodynamics/Wave loads (U>0)/Wave loads U = U1 ==
  eta : Inport
  waves : Inport  Port=2
  U_idx : Inport  Port=3
  Abs : Abs
  Bus Selector : BusSelector  OutputSignals=Psi,Wavenum,Omega,Phase,Zeta_a
  Compare To Constant : simulink/Logic and Bit Operations/Compare To Constant  relop=<  const=0  OutDataTypeStr=uint8  ZeroCross=off
  Conversion : DataTypeConversion  OutDataTypeStr=double  SaturateOnIntegerOverflow=off  RndMeth=Floor
  D2R : Gain  Gain=pi/180
  "D2R " : Gain  Gain=pi/180
  Prelookup [0,180] : PreLookup  BreakpointsData=[0:10:180]  IndexSearchMethod=Evenly spaced points  BeginIndexSearchUsingPreviousIndexResult=on
  Product{,1..3} (4 alike) : Product  RndMeth=Zero
  R2D : Gain  Gain=180/pi
  Selector : Selector  InputPortWidth=6  IndexOptions=Index vector (dialog)  Indices=[6]  OutputSizes=1
  Sign : Signum
  Sum1 : Sum  Inputs=++|
  Sum2 : Sum  Inputs=++|
  Sum4 : Sum  Inputs=-+|
  Sum5 : Sum  Inputs=++|
  Wave loads for heading 1 : $bdroot/Hydrodynamics/Wave loads for heading1  ForceRAO_Freq=vessel.forceRAO.w  WD_Freq=vessel.driftfrc.w  RAO_Vel=vessel.velocities  ForceRAO_Amp=vessel.forceRAO.amp  ForceRAO_Phase=vessel.forceRAO.phase  WD_Amp=vessel.driftfrc.amp  RAO_add_omega_0=on  RAO_add_omega_inf=on
  Wave loads for heading 2 : $bdroot/Hydrodynamics/Wave loads for heading1  ForceRAO_Freq=vessel.forceRAO.w  WD_Freq=vessel.driftfrc.w  RAO_Vel=vessel.velocities  ForceRAO_Amp=vessel.forceRAO.amp  ForceRAO_Phase=vessel.forceRAO.phase  WD_Amp=vessel.driftfrc.amp  RAO_add_omega_0=on  RAO_add_omega_inf=on
  "deg to 180/180 " : $bdroot/Utilities/Math Operations/deg to 180//180
  one : Constant
  "one " : Constant
  psi1 : Subsystem
  psi2 : Subsystem
  tau_WF : Outport
  tau_WD : Outport  Port=2
  wires:
  R2D/1 -> "deg to 180/180 "/1
  Selector/1 -> R2D/1
  Sum5/1 -> tau_WD/1
  waves/1 -> Bus Selector/1
  Sum1/1 -> tau_WF/1
  "D2R "/1 -> Wave loads for heading 2/2
  D2R/1 -> Wave loads for heading 1/2
  psi2/1(psi) -> "D2R "/1
  Conversion/1 -> psi1/1(k), Sum2/2
  Prelookup [0,180]/2 -> Sum4/1, Product1/1, Product3/1
  psi1/1(psi) -> D2R/1
  Compare To Constant/1 -> psi2/2(0 or 1), psi1/2(0 or 1)
  Sign/1 -> Compare To Constant/1
  Abs/1 -> Prelookup [0,180]/1
  "deg to 180/180 "/1 -> Sign/1, Abs/1
  Sum2/1 -> psi2/1(k)
  one/1 -> Sum2/1
  Prelookup [0,180]/1 -> Conversion/1
  Product2/1 -> Sum5/1
  Product3/1 -> Sum5/2
  Wave loads for heading 1/2 -> Product2/2
  Sum4/1 -> Product2/1, Product/1
  "one "/1 -> Sum4/2
  Product1/1 -> Sum1/2
  Product/1 -> Sum1/1
  Wave loads for heading 1/1 -> Product/2
  Bus Selector/5 -> Wave loads for heading 1/7, Wave loads for heading 2/7  "<Zeta_a>"
  Bus Selector/4 -> Wave loads for heading 1/6, Wave loads for heading 2/6  "<Phase>"
  Bus Selector/3 -> Wave loads for heading 1/5, Wave loads for heading 2/5  "<Omega>"
  Bus Selector/2 -> Wave loads for heading 1/4, Wave loads for heading 2/4  "<Wavenum>"
  Bus Selector/1 -> Wave loads for heading 1/3, Wave loads for heading 2/3  "<Psi>"
  eta/1 -> Selector/1, Wave loads for heading 1/1, Wave loads for heading 2/1
  Wave loads for heading 2/2 -> Product3/2
  Wave loads for heading 2/1 -> Product1/2
  U_idx/1 -> Wave loads for heading 1/8, Wave loads for heading 2/8
